simulink model "NUEDC2026A_SVPWM"  (R2024b)
settings: Solver=ode3  StartTime=0.0  StopTime=10.0  FixedStep=Ts_power  RelTol=1e-3
model workspace (MAT data in the model file):
  C_filter = 1e-05
  Io_rms = 2
  L_filter = 0.0011
  P_unmodelled_W = 0
  Ts_power = 1e-06
  Ui_rms = 36
  Ull_rms = 32
  Vdc_ref = 60
  f_out = 60
  fi = 50
  fsw = 20000
libraries: spsSeriesRLCBranchLib x13, spsRMSLib x8, spsCurrentMeasurementLib x5, spsVoltageMeasurementLib x4, spsTHDLib x3, simulink x2, spsMeanLib x2, spsUniversalBridgeLib x2, spsACVoltageSourceLib x1, slpidlib x1, spsPowerLib x1, sps_lib x1
settings Model: SimulationMode=rapid-accelerator  Creator=50803  LastModifiedBy=Lenovo

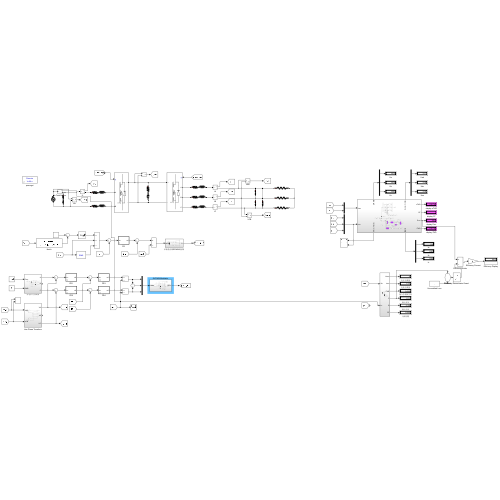
[thumbnail: Simulink's stored preview of the top-level diagram]
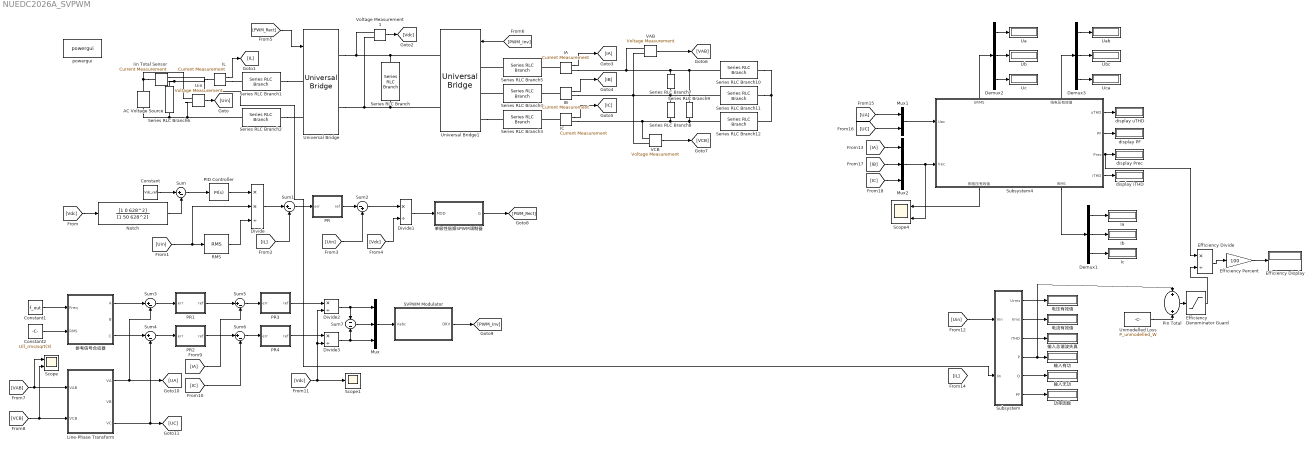
== system NUEDC2026A_SVPWM ==
  AC Voltage Source : spsACVoltageSourceLib/AC Voltage Source  Amplitude=Ui_rms*sqrt(2)  Phase=0  Frequency=fi  SampleTime=0  Measurements=None  BusType=swing  Pref=10e3  Qref=0  Qmin=-inf  Qmax=+inf
  Constant : Constant  Value=Vdc_ref
  Constant1 : Constant  Value=f_out
  Constant2 : Constant  Value=Ull_rms/sqrt(3)
  Demux1 : Demux  Outputs=3
  Demux2 : Demux  Outputs=3
  Demux3 : Demux  Outputs=3
  Divide : Product  Inputs=**/
  Divide1 : Product  Inputs=*/
  Divide2 : Product  Inputs=*/
  Divide3 : Product  Inputs=*/
  Efficiency Denominator Guard : Saturate  UpperLimit=inf  LowerLimit=eps
  Efficiency Display : Display
  Efficiency Divide : Product  Inputs=*/
  Efficiency Percent : Gain  Gain=100
  IA : spsCurrentMeasurementLib/Current Measurement  PhasorSimulation=off  OutputType=Complex  PSBequivalent=0
  IB : spsCurrentMeasurementLib/Current Measurement  PhasorSimulation=off  OutputType=Complex  PSBequivalent=0
  IC : spsCurrentMeasurementLib/Current Measurement  PhasorSimulation=off  OutputType=Complex  PSBequivalent=0
  IL : spsCurrentMeasurementLib/Current Measurement  PhasorSimulation=off  OutputType=Complex  PSBequivalent=0
  Ia : Display
  Ib : Display
  Ic : Display
  Iin Total Sensor : spsCurrentMeasurementLib/Current Measurement  PhasorSimulation=off  OutputType=Complex  PSBequivalent=0
  Line-Phase Transform : Subsystem
  Mux : Mux  Inputs=3
  Mux1 : Mux  Inputs=2
  Mux2 : Mux  Inputs=3
  Notch : TransferFcn  Numerator=[1 0 628^2]  Denominator=[1 50 628^2]
  PID Controller : slpidlib/PID Controller  Controller=PI  Form=Parallel  TimeDomain=Continuous-time  UseExternalTs=off  SampleTime=-1  IntegratorMethod=Forward Euler  FilterMethod=Forward Euler  ControllerParametersSource=internal  P=1  I=1  UseKiTs=off  D=0  UseExternalDerivativeSource=off  N=100  UseFilter=on  TunerSelectOption=Transfer Function Based (PID Tuner App)  InitialConditionSource=internal  InitialConditionForIntegrator=0  InitialConditionForFilter=0  DifferentiatorICPrevScaledInput=0  ExternalReset=none  TrackingMode=off  Kt=1  LimitOutput=on  SatLimitsSource=internal  UpperSaturationLimit=5  LowerSaturationLimit=-5  LinearizeAsGain=on  AntiWindupMode=clamping  Kb=1  LimitIntegrator=off  UpperIntegratorSaturationLimit=inf  LowerIntegratorSaturationLimit=-inf  POutMin=[]  POutMax=[]  IOutMin=[]  IOutMax=[]  DOutMin=[]  DOutMax=[]  NOutMin=[]  NOutMax=[]  SumOutMin=[]  SumOutMax=[]  SaturationOutMin=[]  SaturationOutMax=[]  PParamMin=[]  PParamMax=[]  IParamMin=[]  IParamMax=[]  DParamMin=[]  DParamMax=[]  NParamMin=[]  NParamMax=[]  KbParamMin=[]  KbParamMax=[]  KtParamMin=[]  KtParamMax=[]  KbOutMin=[]  KbOutMax=[]  KtOutMin=[]  KtOutMax=[]  IntegratorOutMin=[]  IntegratorOutMax=[]  FilterOutMin=[]  FilterOutMax=[]  SumI1OutMin=[]  SumI1OutMax=[]  SumI2OutMin=[]  SumI2OutMax=[]  SumI3OutMin=[]  SumI3OutMax=[]  SumI4OutMin=[]  SumI4OutMax=[]  SumDOutMin=[]  SumDOutMax=[]  DifferentiatorOutMin=[]  DifferentiatorOutMax=[]  FilterDiffOutCoefMin=[]  FilterDiffOutCoefMax=[]  ReciprocalOutMin=[]  ReciprocalOutMax=[]  SumDenOutMin=[]  SumDenOutMax=[]  SumNumOutMin=[]  SumNumOutMax=[]  DivideOutMin=[]  DivideOutMax=[]  UdiffTsProdOutMin=[]  UdiffTsProdOutMax=[]  NTsProdOutMin=[]  NTsProdOutMax=[]  UintegralTsProdOutMin=[]  UintegralTsProdOutMax=[]  UngainTsProdOutMin=[]  UngainTsProdOutMax=[]  ClampingZeroOutDataTypeStr=Inherit: Inherit via back propagation  ClampingZeroOutMin=[]  ClampingZeroOutMax=[]  FilterDenConstantOutDataTypeStr=Inherit: Inherit via back propagation  FilterDenConstantOutMin=[]  FilterDenConstantOutMax=[]  PCopyOutDataTypeStr=Inherit: Inherit via back propagation  PCopyOutMin=[]  PCopyOutMax=[]  NCopyOutDataTypeStr=Inherit: Inherit via back propagation  NCopyOutMin=[]  NCopyOutMax=[]  IntegratorContinuousStateAttributes=''  IntegratorStateMustResolveToSignalObject=off  IntegratorRTWStateStorageClass=Auto  FilterContinuousStateAttributes=''  FilterStateMustResolveToSignalObject=off  FilterRTWStateStorageClass=Auto  ParallelPVariant=InternalParameters  IdealPVariant=Disabled  IVariant=InternalParameters  DVariant=Disabled  IntegratorVariant=Continuous  SatVariant=Enabled  AWVariant=ContClampingParallel  PCopyVariant=Disabled  TRVariant=Disabled  FdbkBlocksVariant=Forward  IdealPFdbkVariant=Disabled  SatFdbkVariant=Disabled  DerivativeFilterVariant=Disabled  NVariant=Disabled  NCopyVariant=Disabled_SignalSpec  FilterICVariant=Disabled  IntegratorICVariant=InternalICs  ExternalResetVariant=Disabled  TRSumVariant=Passthrough  SumFdbkVariant=Disabled  SumVariant=Sum_PI  TsampFilterVariant=InternalTs  TsampNgainVariant=Passthrough  TsampIntegralVariant=Disabled_SignalSpec  ExternalSaturationOutDataTypeStr=Inherit: Same as second input  DerivativeSourceVariant=Disabled  PreIntVariant=InternalPreInt
  PR : Subsystem  TreatAsAtomicUnit=on  mask{Kp=5, Kr=60, Wc=5, Wr=2*pi*fi, Upper=1200, Lower=-1200}
  PR1 : Subsystem  TreatAsAtomicUnit=on  mask{Kp=0.05, Kr=30, Wc=1, Wr=2*pi*f_out, Upper=1200, Lower=-1200}
  PR2 : Subsystem  TreatAsAtomicUnit=on  mask{Kp=0.05, Kr=30, Wc=1, Wr=2*pi*f_out, Upper=1200, Lower=-1200}
  PR3 : Subsystem  TreatAsAtomicUnit=on  mask{Kp=5, Kr=60, Wc=5, Wr=2*pi*f_out, Upper=1200, Lower=-1200}
  PR4 : Subsystem  TreatAsAtomicUnit=on  mask{Kp=5, Kr=60, Wc=5, Wr=2*pi*f_out, Upper=1200, Lower=-1200}
  Pin Total : Sum
  RMS : spsRMSLib/RMS  TrueRMS=on  Freq=fi  RMSInit=120  Ts=0
  SVPWM Modulator : Subsystem
  Scope : Scope  NumInputPorts=2
  Scope1 : Scope
  Scope4 : Scope  NumInputPorts=2
  Series RLC Branch : spsSeriesRLCBranchLib/Series RLC Branch  LConnTagsString=__new0  RConnTagsString=__new0  BranchType=RC  Resistance=100e-3  Inductance=1e-3  SetiL0=off  InitialCurrent=0  Capacitance=4400e-6  Setx0=off  InitialVoltage=0  Measurements=None
  Series RLC Branch{1..5} (5 alike) : spsSeriesRLCBranchLib/Series RLC Branch  LConnTagsString=__new0  RConnTagsString=__new0  BranchType=RL  Resistance=100e-3  Inductance=L_filter  SetiL0=off  InitialCurrent=0  Capacitance=4400e-6  Setx0=off  InitialVoltage=0  Measurements=None
  Series RLC Branch10 : spsSeriesRLCBranchLib/Series RLC Branch  LConnTagsString=__new0  RConnTagsString=__new0  BranchType=R  Resistance=Ull_rms/(sqrt(3)*Io_rms)  Inductance=470e-6  SetiL0=off  InitialCurrent=0  Capacitance=4400e-6  Setx0=off  InitialVoltage=0  Measurements=None
  Series RLC Branch11 : spsSeriesRLCBranchLib/Series RLC Branch  LConnTagsString=__new0  RConnTagsString=__new0  BranchType=R  Resistance=Ull_rms/(sqrt(3)*Io_rms)  Inductance=470e-6  SetiL0=off  InitialCurrent=0  Capacitance=4400e-6  Setx0=off  InitialVoltage=0  Measurements=None
  Series RLC Branch12 : spsSeriesRLCBranchLib/Series RLC Branch  LConnTagsString=__new0  RConnTagsString=__new0  BranchType=R  Resistance=Ull_rms/(sqrt(3)*Io_rms)  Inductance=470e-6  SetiL0=off  InitialCurrent=0  Capacitance=4400e-6  Setx0=off  InitialVoltage=0  Measurements=None
  Series RLC Branch6 : spsSeriesRLCBranchLib/Series RLC Branch  LConnTagsString=__new0  RConnTagsString=__new0  BranchType=RC  Resistance=100e-3  Inductance=1e-3  SetiL0=off  InitialCurrent=0  Capacitance=C_filter  Setx0=off  InitialVoltage=0  Measurements=None
  Series RLC Branch7 : spsSeriesRLCBranchLib/Series RLC Branch  LConnTagsString=__new0  RConnTagsString=__new0  BranchType=RC  Resistance=10e-3  Inductance=1e-3  SetiL0=off  InitialCurrent=0  Capacitance=C_filter  Setx0=off  InitialVoltage=0  Measurements=None
  Series RLC Branch8 : spsSeriesRLCBranchLib/Series RLC Branch  LConnTagsString=__new0  RConnTagsString=__new0  BranchType=RC  Resistance=10e-3  Inductance=1e-3  SetiL0=off  InitialCurrent=0  Capacitance=C_filter  Setx0=off  InitialVoltage=0  Measurements=None
  Series RLC Branch9 : spsSeriesRLCBranchLib/Series RLC Branch  LConnTagsString=__new0  RConnTagsString=__new0  BranchType=RC  Resistance=10e-3  Inductance=1e-3  SetiL0=off  InitialCurrent=0  Capacitance=C_filter  Setx0=off  InitialVoltage=0  Measurements=None
  Subsystem : Subsystem
  Subsystem4 : Subsystem
      settings: PortSchema="{\"entries\":[{\"content\":{\"sides\":[{\"content\":{\"connectorIds\":[\"In1\",\"In2\"]},\"type\":\"ConnectorPlacement.EquallySpacedRectSide\",\"uuid\":\"8f3b7bf1-7c44-4492-a357-aa6e3e6d66a4\"},{\"content\":{\"connectorIds\":[\"Out1\",\"Out2\",\"Out3\",\"Out4\"],\"side\":\"RIGHT\"},\"type\":\"ConnectorPlacement.EquallySpacedRectSide\",\"uuid\":\"7ae784cf-6bcf-4684-9c07-1770fc60c8a0\"},{\"content\":{\"connectorIds\":[\"Out7\",\"Out8\"],\"side\":\"TOP\"},\"type\":\"ConnectorPlacement.EquallySpacedRectSide\",\"uuid\":\"0e016931-6232-4ad6-afe9-572a0571336f\"},{\"content\":{\"connectorIds\":[\"Out5\",\"Out6\"],\"side\":\"BOTTOM\"},\"type\":\"ConnectorPlacement.EquallySpacedRectSide\",\"uuid\":\"ef67c6ee-ba81-4705-af34-81581e7e9907\"}]},\"type\":\"ConnectorPlacement.EquallySpacedConnector\",\"uuid\":\"922af512-c0ff-443f-816c-194775a78dc8\"}],\"packageUris\":[\"http://schema.mathworks.com/mf0/Connector/R2020b\"],\"version\":\"1.0\"}"
  Sum{,1,3..6} (6 alike) : Sum  Inputs=|+-
  Sum2 : Sum  Inputs=|-+
  Sum7 : Sum  Inputs=-|-
  Ua : Display
  Uab : Display
  Ub : Display
  Ubc : Display
  Uc : Display
  Uca : Display
  Uin : spsVoltageMeasurementLib/Voltage Measurement  PhasorSimulation=off  OutputType=Complex  PSBequivalent=0
  Universal Bridge : spsUniversalBridgeLib/Universal Bridge  Arms=2  SnubberResistance=1e5  SnubberCapacitance=inf  Device=MOSFET / Diodes  Ron=1e-3  Lon=0  ForwardVoltages="[  0  0  ]"  ForwardVoltage=0  GTOparameters=[ 10e-6 , 20e-6 ]  IGBTparameters=[ 1e-6 , 2e-6 ]  Measurements=None  Measurements_2=None  converterType=Rectifier
  Universal Bridge1 : spsUniversalBridgeLib/Universal Bridge  Arms=3  SnubberResistance=1e5  SnubberCapacitance=inf  Device=MOSFET / Diodes  Ron=1e-3  Lon=0  ForwardVoltages="[  0  0  ]"  ForwardVoltage=0  GTOparameters=[ 10e-6 , 20e-6 ]  IGBTparameters=[ 1e-6 , 2e-6 ]  Measurements=None  Measurements_2=None  converterType=Rectifier
  Unmodelled Loss : Constant  Value=P_unmodelled_W
  VAB : spsVoltageMeasurementLib/Voltage Measurement  PhasorSimulation=off  OutputType=Complex  PSBequivalent=0
  VCB : spsVoltageMeasurementLib/Voltage Measurement  PhasorSimulation=off  OutputType=Complex  PSBequivalent=0
  Voltage Measurement1 : spsVoltageMeasurementLib/Voltage Measurement  PhasorSimulation=off  OutputType=Complex  PSBequivalent=0
  display PF : Display
  display Prec : Display
  display iTHD : Display
  display uTHD : Display
  powergui : sps_lib/powergui  Priority=1  SimulationMode=Discrete  SampleTime=Ts_power  frequency=fi  Iterations=50  frequencyindice=50  Pbase=100e6  ErrMax=1e-4  UnitsV=kV  UnitsW=MW  buscounter=0  FunctionMessages=off  echomessages=off  EnableUseOfTLC=off  CurrentSourceSwitches=off  DisableSnubberDevices=off  DisableRonSwitches=off  DisableVfSwitches=off  DisplayEquations=off  AutomaticDiscreteSolvers=off  SolverType=Tustin/Backward Euler (TBE)  Interpol=off  ExternalGateDelay=off  methode=off  Ts=100  x0status=blocks  SPID=on  SwTol=0  HookPort=off  NonlinearTolerance=1e-4  nMaxIteration=100  ContinueOnMaxIteration=off  RestoreLinks=warning  ResistiveCurrentMeasurement=off  Frange=[0:2:500]  Ylog=off  Xlog=on  ShowGrid=off  save=off  variable=ZData  structure=0  ZoomFFT=off  StartTime=0.0  cycles=1  DisplayStyle=1  fundamental=fi  FreqAxis=off  MaxFrequency=1000  frequencyindicesteady=1  RmsSteady=1  display=off
  功率因数 : Display
  单极性倍频SPWM调制器 : Subsystem
  参考信号合成器 : Subsystem
  电压有效值 : Display
  电流有效值 : Display
  输入总谐波失真 : Display
  输入无功 : Display
  输入有功 : Display
  wires:
  Uin/1 -> [Uin]
  IL/1 -> [IL]
  Voltage Measurement1/1 -> [Vdc]
  IA/1 -> [IA]
  IB/1 -> [IB]
  IC/1 -> [IC]
  VAB/1 -> [VAB]
  VCB/1 -> [VCB]
  Constant/1 -> Sum/1
  [Vdc] -> Notch/1
  Sum/1 -> PID Controller/1
  PID Controller/1 -> Divide/1
  Notch/1 -> Sum/2
  [Uin] -> Divide/2, RMS/1
  RMS/1 -> Divide/3
  Divide/1 -> Sum1/1
  [IL] -> Sum1/2
  Sum1/1 -> PR/1(err)
  PR/1(ref) -> Sum2/1
  [Uin] -> Sum2/2
  Sum2/1 -> Divide1/1
  [Vdc] -> Divide1/2
  Divide1/1 -> 单极性倍频SPWM调制器/1(MOD)
  单极性倍频SPWM调制器/1(G) -> [PWM_Rect]
  [PWM_Rect] -> Universal Bridge/1
  SVPWM Modulator/1(DRV) -> [PWM_Inv]
  [PWM_Inv] -> Universal Bridge1/1
  [VAB] -> Scope/1, Line-Phase Transform/1(VAB)
  [VCB] -> Scope/2, Line-Phase Transform/2(VCB)
  Constant1/1 -> 参考信号合成器/1(Freq)
  Constant2/1 -> 参考信号合成器/2(RMS)
  参考信号合成器/3(C) -> Sum4/1
  参考信号合成器/1(A) -> Sum3/1
  Line-Phase Transform/1(VA) -> [UA], Sum3/2
  Line-Phase Transform/3(VC) -> [UC], Sum4/2
  Sum3/1 -> PR1/1(err)
  Sum4/1 -> PR2/1(err)
  PR2/1(ref) -> Sum6/1
  PR1/1(ref) -> Sum5/1
  [IA] -> Sum5/2
  [IC] -> Sum6/2
  Sum5/1 -> PR3/1(err)
  Sum6/1 -> PR4/1(err)
  [Vdc] -> Divide3/2, Divide2/2, Scope1/1
  Divide2/1 -> Mux/1, Sum7/1
  Divide3/1 -> Sum7/2, Mux/3
  Sum7/1 -> Mux/2
  Mux/1 -> SVPWM Modulator/1(Vabc)
  PR3/1(ref) -> Divide2/1
  PR4/1(ref) -> Divide3/1
  Demux1/3 -> Ic/1
  Demux1/1 -> Ia/1
  Demux1/2 -> Ib/1
  Subsystem4/7(URMS) -> Demux2/1
  Subsystem4/5(相电压有效值) -> Scope4/1
  Subsystem4/1(uTHD) -> display uTHD/1
  Mux1/1 -> Subsystem4/1(Uac)
  Subsystem4/3(Prec) -> display Prec/1, Efficiency Divide/1
  Demux2/1 -> Ua/1
  Demux2/3 -> Uc/1
  Subsystem4/4(iTHD) -> display iTHD/1
  Subsystem4/2(PF) -> display PF/1
  Demux2/2 -> Ub/1
  Subsystem4/6(IRMS) -> Demux1/1
  Mux2/1 -> Scope4/2, Subsystem4/2(Irec)
  [UC] -> Mux1/2
  [UA] -> Mux1/1
  [IC] -> Mux2/3
  [IA] -> Mux2/1
  [IB] -> Mux2/2
  Subsystem/3(iTHD) -> 输入总谐波失真/1
  [Uin] -> Subsystem/1(Vin)
  Subsystem/4(P) -> 输入有功/1, Pin Total/1
  Subsystem/6(PF) -> 功率因数/1
  Subsystem/5(Q) -> 输入无功/1
  Subsystem/2(Irms) -> 电流有效值/1
  Subsystem/1(Urms) -> 电压有效值/1
  Demux3/2 -> Ubc/1
  Demux3/3 -> Uca/1
  Demux3/1 -> Uab/1
  Subsystem4/8(线电压有效值) -> Demux3/1
  Iin Total Sensor/1 -> Subsystem/2(Iin)
  Unmodelled Loss/1 -> Pin Total/2
  Efficiency Divide/1 -> Efficiency Percent/1
  Efficiency Percent/1 -> Efficiency Display/1
  Pin Total/1 -> Efficiency Denominator Guard/1
  Efficiency Denominator Guard/1 -> Efficiency Divide/2
  connections:
  Universal Bridge/RConn2 -- Voltage Measurement1/LConn2 -- Series RLC Branch/RConn1 -- Universal Bridge1/RConn2
  Universal Bridge/RConn1 -- Voltage Measurement1/LConn1 -- Series RLC Branch/LConn1 -- Universal Bridge1/RConn1
  Series RLC Branch1/RConn1 -- Universal Bridge/LConn1
  Series RLC Branch2/RConn1 -- Universal Bridge/LConn2
  Universal Bridge1/LConn3 -- Series RLC Branch3/LConn1
  Series RLC Branch5/LConn1 -- Universal Bridge1/LConn1
  Series RLC Branch4/LConn1 -- Universal Bridge1/LConn2
  IL/RConn1 -- Series RLC Branch1/LConn1
  IA/LConn1 -- Series RLC Branch5/RConn1
  IB/LConn1 -- Series RLC Branch4/RConn1
  IC/LConn1 -- Series RLC Branch3/RConn1
  AC Voltage Source/LConn1 -- Uin/LConn2 -- Series RLC Branch2/LConn1 -- Series RLC Branch6/RConn1
  IA/RConn1 -- VAB/LConn1 -- Series RLC Branch9/LConn1 -- Series RLC Branch10/LConn1 -- Series RLC Branch7/LConn1
  IB/RConn1 -- VCB/LConn2 -- VAB/LConn2 -- Series RLC Branch11/LConn1 -- Series RLC Branch8/LConn1 -- Series RLC Branch7/RConn1
  IC/RConn1 -- VCB/LConn1 -- Series RLC Branch12/LConn1 -- Series RLC Branch9/RConn1 -- Series RLC Branch8/RConn1
  Series RLC Branch10/RConn1 -- Series RLC Branch11/RConn1 -- Series RLC Branch12/RConn1
  Iin Total Sensor/LConn1 -- AC Voltage Source/RConn1 -- Uin/LConn1
  IL/LConn1 -- Iin Total Sensor/RConn1 -- Series RLC Branch6/LConn1

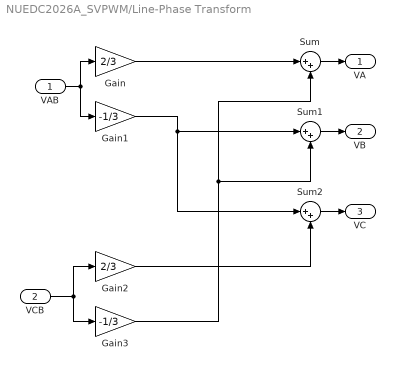
== system NUEDC2026A_SVPWM/Line-Phase Transform ==
  VAB : Inport
  VCB : Inport  Port=2
  Gain : Gain  Gain=2/3
  Gain1 : Gain  Gain=-1/3
  Gain2 : Gain  Gain=2/3
  Gain3 : Gain  Gain=-1/3
  Sum : Sum  Inputs=|++
  Sum1 : Sum  Inputs=|++
  Sum2 : Sum  Inputs=|++
  VA : Outport
  VB : Outport  Port=2
  VC : Outport  Port=3
  wires:
  VCB/1 -> Gain2/1, Gain3/1
  VAB/1 -> Gain/1, Gain1/1
  Sum/1 -> VA/1
  Sum1/1 -> VB/1
  Sum2/1 -> VC/1
  Gain/1 -> Sum/1
  Gain3/1 -> Sum1/2, Sum/2
  Gain1/1 -> Sum2/1, Sum1/1
  Gain2/1 -> Sum2/2

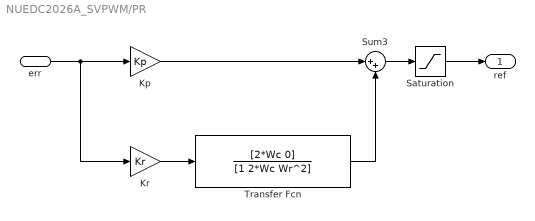
== system NUEDC2026A_SVPWM/PR ==
  err : Inport
  Kp : Gain  Gain=Kp
  Kr : Gain  Gain=Kr
  Saturation : Saturate  UpperLimit=Upper  LowerLimit=Lower
  Sum3 : Sum  Inputs=|++
  Transfer Fcn : TransferFcn  Numerator=[2*Wc 0]  Denominator=[1 2*Wc Wr^2]
  ref : Outport
  wires:
  Kp/1 -> Sum3/1
  Sum3/1 -> Saturation/1
  err/1 -> Kr/1, Kp/1
  Kr/1 -> Transfer Fcn/1
  Transfer Fcn/1 -> Sum3/2
  Saturation/1 -> ref/1

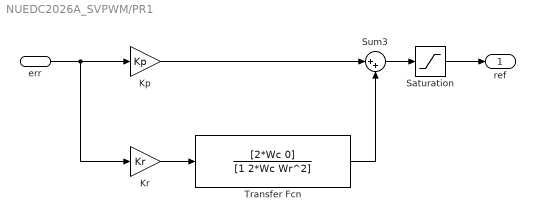
== system NUEDC2026A_SVPWM/PR1 ==
  err : Inport
  Kp : Gain  Gain=Kp
  Kr : Gain  Gain=Kr
  Saturation : Saturate  UpperLimit=Upper  LowerLimit=Lower
  Sum3 : Sum  Inputs=|++
  Transfer Fcn : TransferFcn  Numerator=[2*Wc 0]  Denominator=[1 2*Wc Wr^2]
  ref : Outport
  wires:
  Saturation/1 -> ref/1
  Transfer Fcn/1 -> Sum3/2
  Kr/1 -> Transfer Fcn/1
  err/1 -> Kp/1, Kr/1
  Sum3/1 -> Saturation/1
  Kp/1 -> Sum3/1

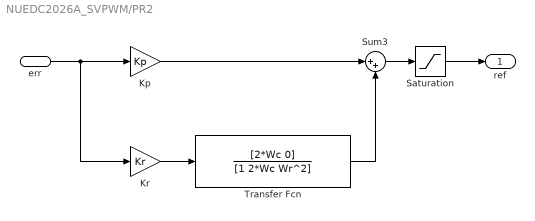
== system NUEDC2026A_SVPWM/PR2 ==
  err : Inport
  Kp : Gain  Gain=Kp
  Kr : Gain  Gain=Kr
  Saturation : Saturate  UpperLimit=Upper  LowerLimit=Lower
  Sum3 : Sum  Inputs=|++
  Transfer Fcn : TransferFcn  Numerator=[2*Wc 0]  Denominator=[1 2*Wc Wr^2]
  ref : Outport
  wires:
  Kp/1 -> Sum3/1
  Sum3/1 -> Saturation/1
  err/1 -> Kr/1, Kp/1
  Kr/1 -> Transfer Fcn/1
  Transfer Fcn/1 -> Sum3/2
  Saturation/1 -> ref/1

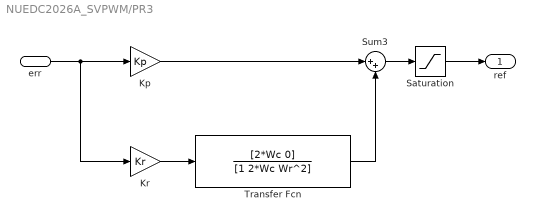
== system NUEDC2026A_SVPWM/PR3 ==
  err : Inport
  Kp : Gain  Gain=Kp
  Kr : Gain  Gain=Kr
  Saturation : Saturate  UpperLimit=Upper  LowerLimit=Lower
  Sum3 : Sum  Inputs=|++
  Transfer Fcn : TransferFcn  Numerator=[2*Wc 0]  Denominator=[1 2*Wc Wr^2]
  ref : Outport
  wires:
  Kp/1 -> Sum3/1
  Sum3/1 -> Saturation/1
  err/1 -> Kr/1, Kp/1
  Kr/1 -> Transfer Fcn/1
  Transfer Fcn/1 -> Sum3/2
  Saturation/1 -> ref/1

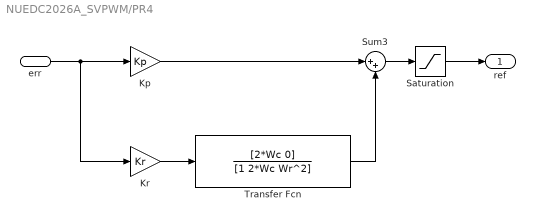
== system NUEDC2026A_SVPWM/PR4 ==
  err : Inport
  Kp : Gain  Gain=Kp
  Kr : Gain  Gain=Kr
  Saturation : Saturate  UpperLimit=Upper  LowerLimit=Lower
  Sum3 : Sum  Inputs=|++
  Transfer Fcn : TransferFcn  Numerator=[2*Wc 0]  Denominator=[1 2*Wc Wr^2]
  ref : Outport
  wires:
  Saturation/1 -> ref/1
  Transfer Fcn/1 -> Sum3/2
  Kr/1 -> Transfer Fcn/1
  err/1 -> Kp/1, Kr/1
  Sum3/1 -> Saturation/1
  Kp/1 -> Sum3/1

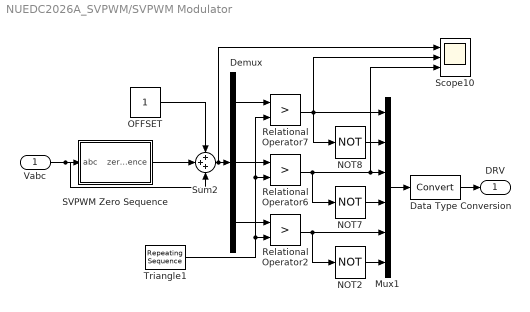
== system NUEDC2026A_SVPWM/SVPWM Modulator ==
  Vabc : Inport
  Data Type Conversion : DataTypeConversion  SaturateOnIntegerOverflow=off  RndMeth=Floor
  Demux : Demux  Outputs=3
  Mux1 : Mux  Inputs=6
  NOT2 : Logic  Operator=NOT  IconShape=distinctive  AllPortsSameDT=off  OutDataTypeStr=boolean
  NOT7 : Logic  Operator=NOT  IconShape=distinctive  AllPortsSameDT=off  OutDataTypeStr=boolean
  NOT8 : Logic  Operator=NOT  IconShape=distinctive  AllPortsSameDT=off  OutDataTypeStr=boolean
  OFFSET : Constant
  Relational Operator2 : RelationalOperator  Operator=>  OutDataTypeStr=boolean  InputSameDT=off
  Relational Operator6 : RelationalOperator  Operator=>  OutDataTypeStr=boolean  InputSameDT=off
  Relational Operator7 : RelationalOperator  Operator=>  OutDataTypeStr=boolean  InputSameDT=off
  SVPWM Zero Sequence : Subsystem
  Scope10 : Scope  NumInputPorts=3
  Sum2 : Sum  Inputs=+++
  Triangle1 : simulink/Sources/Repeating Sequence  rep_seq_t=[0 1/fsw/2 1/fsw]  rep_seq_y=[0 2 0]
  DRV : Outport
  wires:
  OFFSET/1 -> Sum2/1
  Data Type Conversion/1 -> DRV/1
  Mux1/1 -> Data Type Conversion/1
  Sum2/1 -> Demux/1, Scope10/1
  Demux/3 -> Relational Operator2/1
  Demux/2 -> Relational Operator6/1
  Demux/1 -> Relational Operator7/1
  NOT2/1 -> Mux1/6
  Relational Operator2/1 -> NOT2/1, Mux1/5
  NOT8/1 -> Mux1/2
  Triangle1/1 -> Relational Operator6/2, Relational Operator7/2, Relational Operator2/2
  Relational Operator7/1 -> Mux1/1, Scope10/2, NOT8/1
  NOT7/1 -> Mux1/4
  Relational Operator6/1 -> NOT7/1, Mux1/3, Scope10/3
  Vabc/1 -> Sum2/3, SVPWM Zero Sequence/1(abc)
  SVPWM Zero Sequence/1(zero_sequence) -> Sum2/2

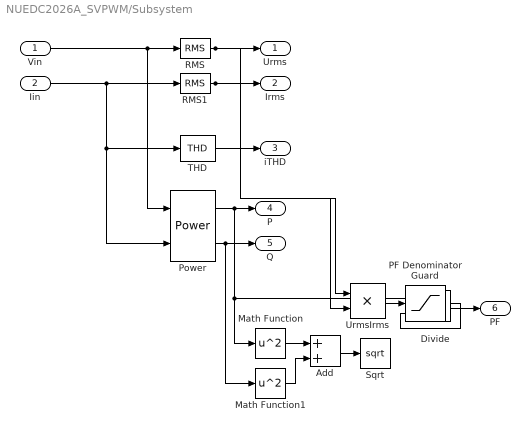
== system NUEDC2026A_SVPWM/Subsystem ==
  Vin : Inport
  Iin : Inport  Port=2
  Add : Sum
  Divide : Product  Inputs=*/
  Math Function : Math  Operator=square
  Math Function1 : Math  Operator=square
  PF Denominator Guard : Saturate  UpperLimit=inf  LowerLimit=eps
  Power : spsPowerLib/Power  Freq=fi  Vinit=[1, 0]  Iinit=[1, 0]  Ts=0
  RMS : spsRMSLib/RMS  TrueRMS=on  Freq=fi  RMSInit=0  Ts=0
  RMS1 : spsRMSLib/RMS  TrueRMS=on  Freq=fi  RMSInit=0  Ts=0
  Sqrt : Sqrt
  THD : spsTHDLib/THD  Freq=fi  Ts=0
  UrmsIrms : Product  Inputs=**
  Urms : Outport
  Irms : Outport  Port=2
  iTHD : Outport  Port=3
  P : Outport  Port=4
  Q : Outport  Port=5
  PF : Outport  Port=6
  wires:
  Iin/1 -> Power/2, THD/1, RMS1/1
  Vin/1 -> Power/1, RMS/1
  RMS/1 -> Urms/1, UrmsIrms/1
  RMS1/1 -> Irms/1, UrmsIrms/2
  THD/1 -> iTHD/1
  Power/1 -> Divide/1, Math Function/1, P/1
  Power/2 -> Math Function1/1, Q/1
  Add/1 -> Sqrt/1
  Math Function/1 -> Add/1
  Math Function1/1 -> Add/2
  Divide/1 -> PF/1
  UrmsIrms/1 -> PF Denominator Guard/1
  PF Denominator Guard/1 -> Divide/2

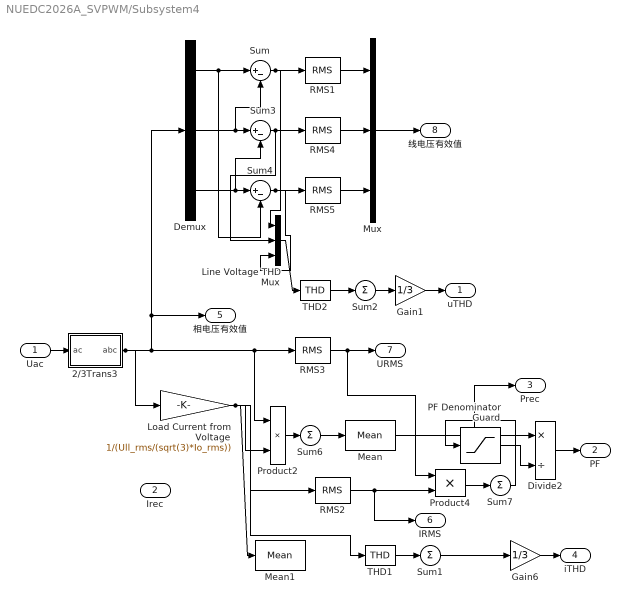
== system NUEDC2026A_SVPWM/Subsystem4 ==
  Uac : Inport
  Irec : Inport  Port=2
  2/3Trans3 : Subsystem
  Demux : Demux  Outputs=3
  Divide2 : Product  Inputs=*/
  Gain1 : Gain  Gain=1/3
  Gain6 : Gain  Gain=1/3
  Line Voltage THD Mux : Mux  Inputs=3
  Load Current from Voltage : Gain  Gain=1/(Ull_rms/(sqrt(3)*Io_rms))
  Mean : spsMeanLib/Mean  Freq=f_out  Vinit=0  Ts=0
  Mean1 : spsMeanLib/Mean  Freq=5000  Vinit=0  Ts=0
  Mux : Mux  Inputs=3
  PF Denominator Guard : Saturate  UpperLimit=inf  LowerLimit=eps
  Product2 : Product
  Product4 : Product
  RMS{1..5} (5 alike) : spsRMSLib/RMS  TrueRMS=on  Freq=f_out  RMSInit=0  Ts=0
  Sum : Sum  Inputs=|+-
  Sum{1..2,6..7} (4 alike) : Sum  Inputs=+
  Sum3 : Sum  Inputs=|+-
  Sum4 : Sum  Inputs=|+-
  THD1 : spsTHDLib/THD  Freq=f_out  Ts=0
  THD2 : spsTHDLib/THD  Freq=f_out  Ts=0
  uTHD : Outport
  PF : Outport  Port=2
  Prec : Outport  Port=3
  iTHD : Outport  Port=4
  相电压有效值 : Outport  Port=5
  IRMS : Outport  Port=6
  URMS : Outport  Port=7
  线电压有效值 : Outport  Port=8
  wires:
  Product2/1 -> Sum6/1
  2/3Trans3/1(abc) -> Product2/1, RMS3/1, 相电压有效值/1, Demux/1, Load Current from Voltage/1
  Uac/1 -> 2/3Trans3/1(ac)
  Product4/1 -> Sum7/1
  RMS3/1 -> URMS/1, Product4/1
  THD1/1 -> Sum1/1
  RMS2/1 -> IRMS/1, Product4/2
  Divide2/1 -> PF/1
  Sum6/1 -> Mean/1
  Gain6/1 -> iTHD/1
  Mean/1 -> Divide2/1, Prec/1
  Sum1/1 -> Gain6/1
  THD2/1 -> Sum2/1
  Sum2/1 -> Gain1/1
  Gain1/1 -> uTHD/1
  Mux/1 -> 线电压有效值/1
  Demux/1 -> Sum4/2, Sum/1
  Sum/1 -> RMS1/1, Line Voltage THD Mux/1
  Demux/2 -> Sum/2, Sum3/1
  Demux/3 -> Sum4/1, Sum3/2
  Sum4/1 -> RMS5/1, Line Voltage THD Mux/3
  Sum3/1 -> RMS4/1, Line Voltage THD Mux/2
  RMS1/1 -> Mux/1
  RMS4/1 -> Mux/2
  RMS5/1 -> Mux/3
  Load Current from Voltage/1 -> Mean1/1, Product2/2, RMS2/1, THD1/1
  Line Voltage THD Mux/1 -> THD2/1
  Sum7/1 -> PF Denominator Guard/1
  PF Denominator Guard/1 -> Divide2/2

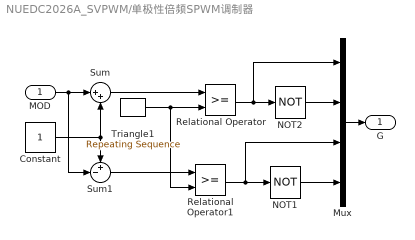
== system NUEDC2026A_SVPWM/单极性倍频SPWM调制器 ==
  MOD : Inport
  Constant : Constant
  Mux : Mux
  NOT1 : Logic  Operator=NOT  IconShape=distinctive  AllPortsSameDT=off  OutDataTypeStr=boolean
  NOT2 : Logic  Operator=NOT  IconShape=distinctive  AllPortsSameDT=off  OutDataTypeStr=boolean
  Relational Operator : RelationalOperator  OutDataTypeStr=boolean  RndMeth=Simplest  InputSameDT=off
  Relational Operator1 : RelationalOperator  OutDataTypeStr=boolean  RndMeth=Simplest  InputSameDT=off
  Sum : Sum  Inputs=|++
  Sum1 : Sum  Inputs=+-|
  Triangle1 : simulink/Sources/Repeating Sequence  rep_seq_t=[0 1/fsw/2 1/fsw]  rep_seq_y=[0 2 0]
  G : Outport
  wires:
  NOT2/1 -> Mux/2
  NOT1/1 -> Mux/4
  Relational Operator1/1 -> NOT1/1, Mux/3
  Sum1/1 -> Relational Operator1/1
  Relational Operator/1 -> Mux/1, NOT2/1
  Triangle1/1 -> Relational Operator/2, Relational Operator1/2
  Sum/1 -> Relational Operator/1
  Constant/1 -> Sum1/1, Sum/2
  Mux/1 -> G/1
  MOD/1 -> Sum/1, Sum1/2

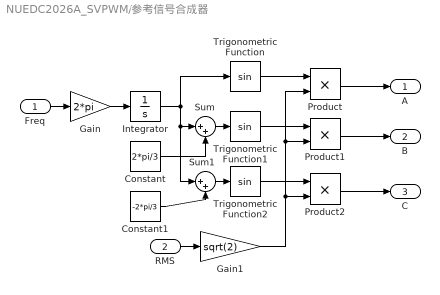
== system NUEDC2026A_SVPWM/参考信号合成器 ==
  Freq : Inport
  RMS : Inport  Port=2
  Constant : Constant  Value=2*pi/3
  Constant1 : Constant  Value=-2*pi/3
  Gain : Gain  Gain=2*pi
  Gain1 : Gain  Gain=sqrt(2)
  Integrator : Integrator  WrapState=on  WrappedStateUpperValue=2*pi  WrappedStateLowerValue=0
  Product : Product
  Product1 : Product
  Product2 : Product
  Sum : Sum  Inputs=|++
  Sum1 : Sum  Inputs=|++
  Trigonometric Function : Trigonometry
  Trigonometric Function1 : Trigonometry
  Trigonometric Function2 : Trigonometry
  A : Outport
  B : Outport  Port=2
  C : Outport  Port=3
  wires:
  Sum/1 -> Trigonometric Function1/1
  Constant/1 -> Sum/2
  Integrator/1 -> Sum1/1, Sum/1, Trigonometric Function/1
  Freq/1 -> Gain/1
  Gain/1 -> Integrator/1
  Constant1/1 -> Sum1/2
  Trigonometric Function/1 -> Product/1
  Trigonometric Function1/1 -> Product1/1
  Trigonometric Function2/1 -> Product2/1
  RMS/1 -> Gain1/1
  Product2/1 -> C/1
  Product1/1 -> B/1
  Product/1 -> A/1
  Gain1/1 -> Product2/2, Product1/2, Product/2
  Sum1/1 -> Trigonometric Function2/1

== system NUEDC2026A_SVPWM/SVPWM Modulator/SVPWM Zero Sequence ==
  abc : Inport
  Demux : Demux  Outputs=3
  Max : MinMax  Function=max  Inputs=3
  MaxPlusMin : Sum
  Min : MinMax  Inputs=3
  MinusHalf : Gain  Gain=-0.5
  zero_sequence : Outport
  wires:
  abc/1 -> Demux/1
  Demux/1 -> Max/1, Min/1
  Demux/2 -> Max/2, Min/2
  Demux/3 -> Max/3, Min/3
  Max/1 -> MaxPlusMin/1
  Min/1 -> MaxPlusMin/2
  MaxPlusMin/1 -> MinusHalf/1
  MinusHalf/1 -> zero_sequence/1

== system NUEDC2026A_SVPWM/Subsystem4/2//3Trans3 ==
  ac : Inport
  Demux2 : Demux  Outputs=2
  Mux1 : Mux  Inputs=3
  Sum2 : Sum  Inputs=-|-
  abc : Outport
  wires:
  ac/1 -> Demux2/1
  Mux1/1 -> abc/1
  Demux2/2 -> Mux1/3, Sum2/2
  Demux2/1 -> Mux1/1, Sum2/1
  Sum2/1 -> Mux1/2
